simulink model "Lab2_VM_Task_5678"  (R2026a)
settings: Solver=FixedStepAuto  StopTime=inf
model workspace (MAT data in the model file):
  SL_ROS_VariableLengthArrays_MaxSizes.CommonInfo.ArrayTruncateAction = 'EmitWarning'
  SL_ROS_VariableLengthArrays_MaxSizes.MsgTypeMap = containers.Map
  SL_ROS_VariableLengthArrays_MaxSizes.MsgTypeMap.serialization.keys = {'sensor_msgs/LaserScan'}
  SL_ROS_VariableLengthArrays_MaxSizes.MsgTypeMap.serialization.values{1}(1).PropertyName = 'Intensities'
  SL_ROS_VariableLengthArrays_MaxSizes.MsgTypeMap.serialization.values{1}(1).DataType = 'single'
  SL_ROS_VariableLengthArrays_MaxSizes.MsgTypeMap.serialization.values{1}(1).MaxLength = 360
  SL_ROS_VariableLengthArrays_MaxSizes.MsgTypeMap.serialization.values{1}(2).PropertyName = 'Ranges'
  SL_ROS_VariableLengthArrays_MaxSizes.MsgTypeMap.serialization.values{1}(2).DataType = 'single'
  SL_ROS_VariableLengthArrays_MaxSizes.MsgTypeMap.serialization.values{1}(2).MaxLength = 360
  SL_ROS_VariableLengthArrays_MaxSizes.MsgTypeMap.serialization.uniformity = 0
  SL_ROS_VariableLengthArrays_MaxSizes.MsgTypeMap.serialization.keyType = 'char'
  SL_ROS_VariableLengthArrays_MaxSizes.MsgTypeMap.serialization.valueType = 'any'
undefined symbols (not defined in the file or in its folder): Angular, Linear
libraries: robotlib x4
settings Model: Creator=Sina  LastModifiedBy=juulg
settings HardwareCC: ProdHWDeviceType=Generic->Unspecified (assume 32-bit Generic)  UseEmbeddedCoderFeatures=off
settings RTWCC: SystemTargetFile=ert.tlc  HardwareBoard=Robot Operating System (ROS)  TLCOptions="-aInlineSetEventsForThisBaseRateFcn=TLC_FALSE -aSuppressMultiTaskScheduler=TLC_FALSE  -aRateBasedStepFcn=0"  Toolchain=Catkin  TargetLang=C++  Description=Embedded Coder
settings ERTTargetCC: SupportNonInlinedSFcns=on

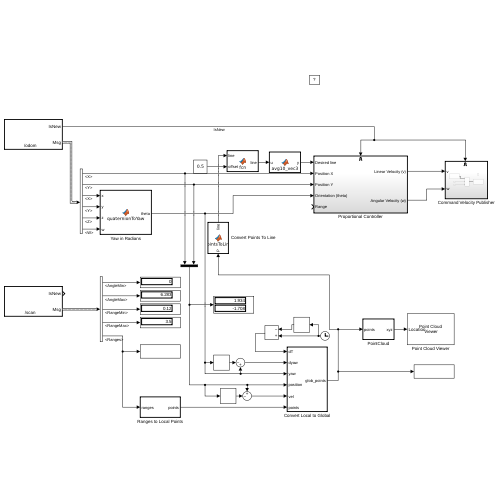
[thumbnail: Simulink's stored preview of the top-level diagram]
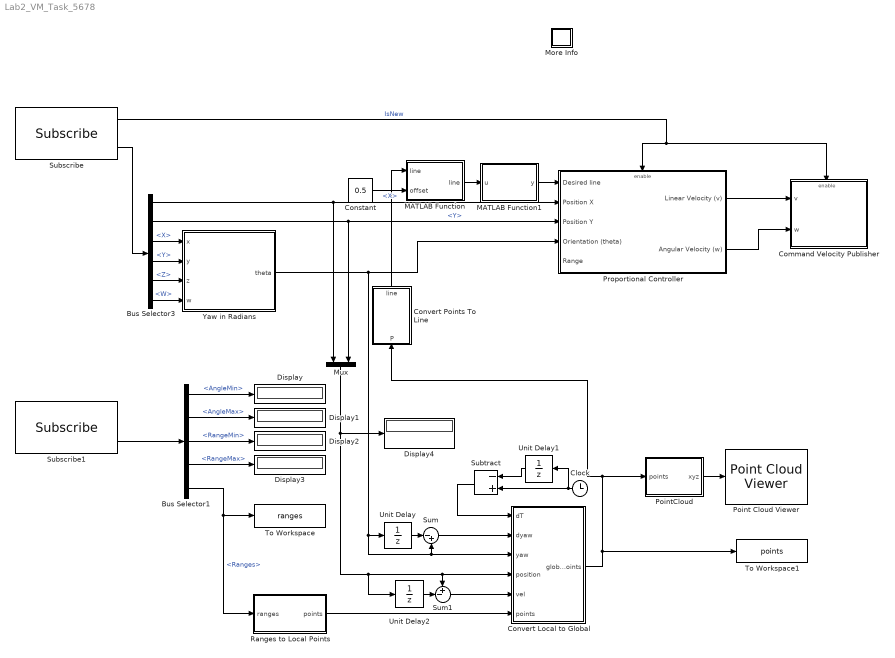
== system Lab2_VM_Task_5678 ==
  Bus Selector1 : BusSelector  OutputSignals=AngleMin,AngleMax,RangeMin,RangeMax,Ranges
  Bus Selector3 : BusSelector  OutputSignals=Pose.Pose.Position.X,Pose.Pose.Position.Y,Pose.Pose.Orientation.X,Pose.Pose.Orientation.Y,Pose.Pose.Orientation.Z,Pose.Pose.Orientation.W
  Clock : Clock
  Command Velocity Publisher : Subsystem
  Constant : Constant  Value=0.5
  Convert Local to Global : MATLAB Function  TreatAsAtomicUnit=on
  Convert Points To Line : MATLAB Function  TreatAsAtomicUnit=on
  Display{,1..4} (5 alike) : Display
      Display settings: Decimation=3
      Display1 settings: Decimation=3
      Display2 settings: Decimation=3
      Display3 settings: Decimation=3
  MATLAB Function : MATLAB Function  TreatAsAtomicUnit=on
  MATLAB Function1 : MATLAB Function  TreatAsAtomicUnit=on
  More Info : Subsystem
      settings: OpenFcn=showdemo(bdroot(gcb))
      mask Display: disp('?')
  Mux : Mux  Inputs=2
  Point Cloud Viewer : PointCloudViewer  FigPos=[3843 1177 1916 1112]  FigSettingsValue=[-7.58662079218697 28.9349744574912 -10.400794325611 5.29998510606108 -1 1 1]
  PointCloud : MATLAB Function  TreatAsAtomicUnit=on
  Proportional Controller : Subsystem
  Ranges to Local Points : MATLAB Function  TreatAsAtomicUnit=on
  Subscribe : robotlib/Subscribe  topicSource=Select from ROS network  topic=/odom  messageType=nav_msgs/Odometry  SampleTime=-1  legacyBusStruct=off  messageQueueLength=51
  Subscribe1 : robotlib/Subscribe  topicSource=Select from ROS network  topic=/scan  messageType=sensor_msgs/LaserScan  SampleTime=-1  legacyBusStruct=off  messageQueueLength=51
  Subtract : Sum  Inputs=-+
  Sum : Sum  Inputs=|-+
  Sum1 : Sum  Inputs=+-|
  To Workspace : ToWorkspace  VariableName=ranges  SaveFormat=Timeseries  SampleTime=-1
  To Workspace1 : ToWorkspace  VariableName=points  SaveFormat=Timeseries  SampleTime=-1
  Unit Delay : UnitDelay  SampleTime=-1
  Unit Delay1 : UnitDelay  SampleTime=-1
  Unit Delay2 : UnitDelay  SampleTime=-1
  Yaw in Radians : MATLAB Function  TreatAsAtomicUnit=on
  wires:
  Proportional Controller/2(Angular Velocity (w)) -> Command Velocity Publisher/2(w)
  Subscribe/1 -> Command Velocity Publisher/Enable, Proportional Controller/Enable  "IsNew"
  Proportional Controller/1(Linear Velocity (v)) -> Command Velocity Publisher/1(v)
  Subscribe/2 -> Bus Selector3/1
  Bus Selector1/5 -> Ranges to Local Points/1(ranges), To Workspace/1  "<Ranges>"
  Subscribe1/2 -> Bus Selector1/1
  Bus Selector1/1 -> Display/1  "<AngleMin>"
  Bus Selector3/3 -> Yaw in Radians/1(x)  "<X>"
  Bus Selector3/4 -> Yaw in Radians/2(y)  "<Y>"
  Bus Selector3/5 -> Yaw in Radians/3(z)  "<Z>"
  Bus Selector3/6 -> Yaw in Radians/4(w)  "<W>"
  Bus Selector3/1 -> Proportional Controller/2(Position X), Mux/1  "<X>"
  Bus Selector3/2 -> Proportional Controller/3(Position Y), Mux/2  "<Y>"
  Bus Selector1/2 -> Display1/1  "<AngleMax>"
  Bus Selector1/4 -> Display3/1  "<RangeMax>"
  Bus Selector1/3 -> Display2/1  "<RangeMin>"
  Yaw in Radians/1(theta) -> Proportional Controller/4(Orientation (theta)), Sum/2, Convert Local to Global/3(yaw), Unit Delay/1
  Ranges to Local Points/1(points) -> Convert Local to Global/6(points)
  Convert Local to Global/1(glob_points) -> PointCloud/1(points), Convert Points To Line/1(P), To Workspace1/1
  PointCloud/1(xyz) -> Point Cloud Viewer/1
  Unit Delay/1 -> Sum/1
  Clock/1 -> Subtract/2, Unit Delay1/1
  Sum/1 -> Convert Local to Global/2(dyaw)
  Unit Delay1/1 -> Subtract/1
  Subtract/1 -> Convert Local to Global/1(dT)
  Unit Delay2/1 -> Sum1/2
  Sum1/1 -> Convert Local to Global/5(vel)
  Mux/1 -> Unit Delay2/1, Sum1/1, Convert Local to Global/4(position), Display4/1
  Convert Points To Line/1(line) -> MATLAB Function/1("line ")
  MATLAB Function/1(line) -> MATLAB Function1/1(u)
  Constant/1 -> MATLAB Function/2(offset)
  MATLAB Function1/1(y) -> Proportional Controller/1(Desired line)

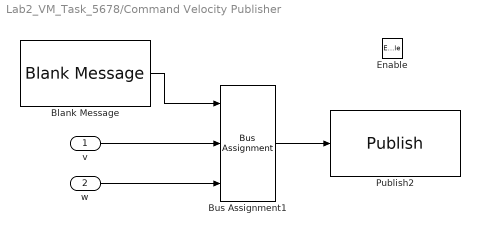
== system Lab2_VM_Task_5678/Command Velocity Publisher ==
  v : Inport
  w : Inport  Port=2
  Enable : EnablePort
  Blank Message : robotlib/Blank Message  messageClass=Message  entityType=geometry_msgs/Twist  messageType=geometry_msgs/Twist  SampleTime=inf  legacyBusStruct=off
  Bus Assignment1 : BusAssignment  DialogController=Simulink.DDGSource_BusAssignment  AssignedSignals=Linear.X,Angular.Z
  Publish2 : robotlib/Publish  topicSource=Select from ROS network  topic=/cmd_vel  messageType=geometry_msgs/Twist  legacyBusStruct=off  messageQueueLength=105
  wires:
  Bus Assignment1/1 -> Publish2/1
  Blank Message/1 -> Bus Assignment1/1
  v/1 -> Bus Assignment1/2
  w/1 -> Bus Assignment1/3

== system Lab2_VM_Task_5678/More Info ==

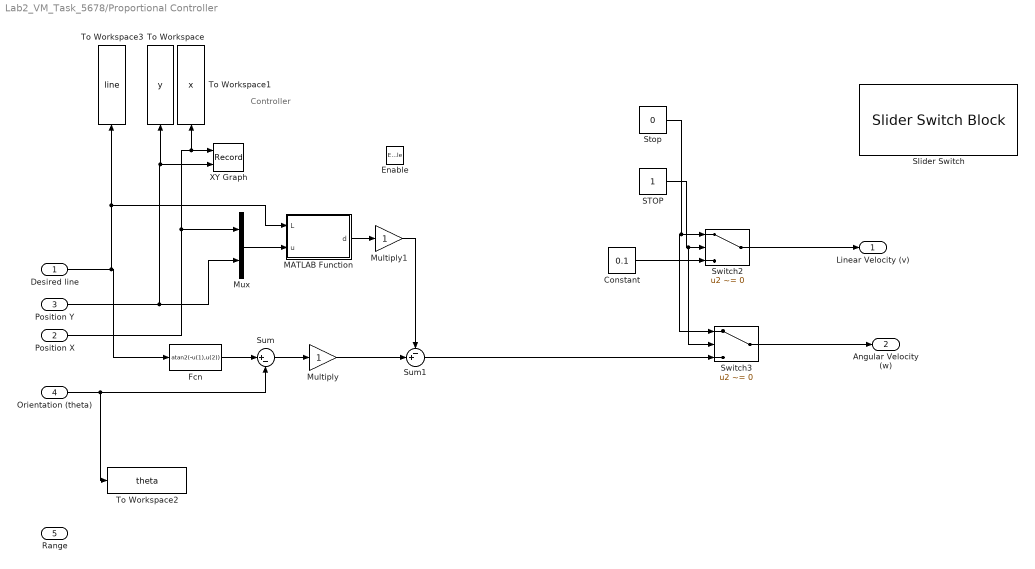
== system Lab2_VM_Task_5678/Proportional Controller ==
  note: Controller
  Desired line : Inport
  Position X : Inport  Port=2
  Position Y : Inport  Port=3
  Orientation (theta) : Inport  Port=4
  Range : Inport  Port=5
  Enable : EnablePort
  Constant : Constant  Value=0.1
  Fcn : Fcn  Expr=atan2(-u(1),u(2))
  MATLAB Function : MATLAB Function  TreatAsAtomicUnit=on
  Multiply : Gain
  Multiply1 : Gain
  Mux : Mux  Inputs=2
  "STOP " : Constant
  Slider Switch : SliderSwitchBlock
  Stop : Constant  Value=0
  Sum : Sum  Inputs=|+-
  Sum1 : Sum  Inputs=-+|
  Switch2 : Switch  Criteria=u2 ~= 0  SaturateOnIntegerOverflow=off  InputSameDT=off
  Switch3 : Switch  Criteria=u2 ~= 0  SaturateOnIntegerOverflow=off  InputSameDT=off
  To Workspace : ToWorkspace  VariableName=y  SaveFormat=Timeseries  SampleTime=-1
  To Workspace1 : ToWorkspace  VariableName=x  SaveFormat=Timeseries  SampleTime=-1
  To Workspace2 : ToWorkspace  VariableName=theta  SaveFormat=Timeseries  SampleTime=-1
  To Workspace3 : ToWorkspace  VariableName=line  SaveFormat=Timeseries  SampleTime=-1
  XY Graph : Record  NumPorts=2.0  FileSettingsInternal="{\"entries\":[{\"content\":{\"excelSettings\":{\"content\":{},\"type\":\"Streamout.ExcelSettings\"},\"parquetSettings\":{\"content\":{},\"type\":\"Streamout.ParquetSettings\"}},\"type\":\"Streamout.FileSettingStorage\",\"uuid\":\"\"}],\"packageUris\":[\"http:\\/\\/schema.mathworks.com\\/mf0\\/streamout_blocks\\/R2020a\"],\"version\":\"1.0\"}"  FrameSettings=[0, 0]  Layout=[1 1]  SignalsInternal="{\"entries\":[{\"content\":{\"signals\":[{\"content\":{\"blockPath\":[],\"dimensions\":[1],\"domain\":\"\",\"lineColor\":\"#a2142f\",\"plots\":[ 1 ],\"port\":1,\"sid\":[\"\"],\"signalID\":1,\"signalName\":\"X\"},\"type\":\"RecordBlkView.Signal\",\"uuid\":\"\"},{\"content\":{\"blockPath\":[],\"dimensions\":[1],\"domain\":\"\",\"lineColor\":\"#139fff\",\"plots\":[ 1 ],\"port\":2,\"sid\":[\"\"],\"signalID\":2,\"signalName\":\"Y\"},\"type\":\"RecordBlkView.Signal\",\"uuid\":\"\"}]},\"type\":\"RecordBlkView.InputSignals\",\"uuid\":\"\"}],\"packageUris\":[\"http:\\/\\/schema.mathworks.com\\/mf0\\/streamout_blocks\\/R2020a\"],\"version\":\"1.0\"}"  VisualizationBindings="{\"xyplotplugin\":{\"info\":[{\"series\":[{\"bindingParametersList\":[{\"parameter\":\"X-Axis\",\"signalID\":1,\"signalName\":\"X\"},{\"parameter\":\"Y-Axis\",\"signalID\":2,\"signalName\":\"Y\"}],\"seriesID\":0}],\"subplotID\":1}]}}"  CompatibilityTag=XY
  Linear Velocity (v) : Outport  VectorParamsAs1DForOutWhenUnconnected=off
  Angular Velocity (w) : Outport  Port=2  VectorParamsAs1DForOutWhenUnconnected=off
  wires:
  Stop/1 -> Switch3/1, Switch2/1
  "STOP "/1 -> Switch3/2, Switch2/2
  Switch2/1 -> Linear Velocity (v)/1
  Switch3/1 -> Angular Velocity (w)/1
  Mux/1 -> MATLAB Function/2(u)
  Multiply1/1 -> Sum1/1
  Position Y/1 -> To Workspace/1, XY Graph/2, Mux/2
  Position X/1 -> Mux/1, To Workspace1/1, XY Graph/1
  Desired line/1 -> Fcn/1, MATLAB Function/1(L), To Workspace3/1
  Sum/1 -> Multiply/1
  Multiply/1 -> Sum1/2
  Fcn/1 -> Sum/1
  Sum1/1 -> Switch3/3
  MATLAB Function/1(d) -> Multiply1/1
  Orientation (theta)/1 -> To Workspace2/1, Sum/2
  Constant/1 -> Switch2/3

== matlab function Lab2_VM_Task_5678/PointCloud ==
  data: points input; xyz output
function xyz = PointCloud(points)
xyz = [points, zeros(size(points, 1), 1)];
end

== matlab function Lab2_VM_Task_5678/Convert Local to Global ==
  data: dT input; dyaw input; yaw input; position input; vel input; points input; glob_points output
function glob_points = LocToGlob(dT, dyaw, yaw, position, vel, points)
% yaw          : heading at START of scan [rad]
% dyaw         : yaw rate [rad/s] (assumed constant over the scan)
% position     : [x y] at START of scan
% vel          : [vx vy] global velocity [m/s] (use [0 0] to ignore)
% points       : N x 2 local lidar points, ordered by measurement time
% T            : scan period [s]

N = size(points,1);
t = linspace(0, dT, N)';                 % time of each point [s]

theta = yaw(1) + dyaw(1) * t;           % heading per point
c = cos(theta);  s = sin(theta);

p = points;

gx = c .* p(:,1) - s .* p(:,2);
gy = s .* p(:,1) + c .* p(:,2);

pos_i = position(:)' + t * vel(:)';     % position per point (N x 2)

glob_points = [gx gy] + pos_i;
end

== matlab function Lab2_VM_Task_5678/Yaw in Radians ==
  data: x input; theta output; y input; z input; w input
function theta = quaternionToYaw(x,y,z,w)

    theta = atan2(2*(w*z + x*y), ...
                  1 - 2*(y*y + z*z));

end

== matlab function Lab2_VM_Task_5678/Ranges to Local Points ==
  data: ranges input; points output
function points = point_cloud(ranges)
l=length(ranges);
points = nan(l, 2);
for i = 1:l
    %if isinf(ranges(i))
    %    continue
    %end
    %angle = (i/l)*(2*pi);
    %x = ranges(i)* cos(angle);
    %y = ranges(i) * sin(angle);
    %points(i) = [x y];
    if ~isinf(ranges(i))
        angle = (i/l) * 2*pi;
        points(i,:) = [ranges(i)*cos(angle), ...
            ranges(i)*sin(angle)];
    end
end

== matlab function Lab2_VM_Task_5678/Convert Points To Line ==
  data: P input; line output
function line = PointsToLine(P)
% Remove rows containing NaN or Inf
P = P(all(isfinite(P),2),:);

% 1. Calculate centroid
C = mean(P,1);

% 2. PCA
[coeff,~,~] = pca(P);

% Direction vector of fitted line
v = coeff(:,1);

% 3. Normal vector to the line
n = [-v(2); v(1)];

% 4. Calculate a, b, c
a = n(1);
b = n(2);
c = -n' * C';

% Normalize coefficients (optional)
s = sqrt(a^2 + b^2);
a = a/s;
b = b/s;
c = c/s;
line = [a b c];

== matlab function Lab2_VM_Task_5678/Proportional Controller/MATLAB Function ==
  data: L input; u input; d output
function d = LineDist(L,u)
d= (u(1)*L(1)+u(2)*L(2)+L(3))/sqrt(L(1)^2+L(2)^2);

== matlab function Lab2_VM_Task_5678/MATLAB Function ==
  data: line input; line output; offset input
function line = fcn(line, offset)
line(3) = line(3)-offset* sqrt(line(1)^2+line(2)^2);

== matlab function Lab2_VM_Task_5678/MATLAB Function1 ==
  data: u input; y output
function y = avg10_vec3(u)
% u must be a 3x1 column vector
persistent buf idx count
if isempty(buf)
    buf = zeros(3, 10);
    idx = 1;
    count = 0;
end
buf(:, idx) = u(:);
idx = mod(idx, 10) + 1;
count = min(count + 1, 10);
y = sum(buf(:, 1:count), 2) / count;
end
